simulink model "grid_forming_dqctrl"  (R2026b)
settings: Solver=VariableStepAuto
undefined symbols (not defined in the file or in its folder): param
libraries: nesl_utility x2, afe_ssc_lib x1
(part 1 of 2)
settings Model: Creator=d.bagnara  LastModifiedBy=dbagn

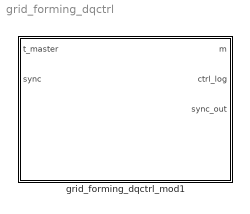
== system grid_forming_dqctrl ==
  grid_forming_dqctrl_mod1 : Subsystem  mask(Grid-forming AFE (two-level bridge, LCL filter)){p=param.afe_mod(1)}
      mask prompts: p "Parameter struct p (afe_module_param)"
      mask help: Grid-forming AFE in one block: ideal two-level bridge, DC-link capacitor and LCL filter as a Simscape language component (afe_ssc.afe_two_level_lcl), control and PWM as one MATLAB Function (afe_dq_ctrl_pwm, source private/afe_dq_ctrl_pwm.m of the library folder), measurements to the control through a Unit Delay of one tc (no algebraic loop). Interface of afe_dq_mod1 of grid_forming_dq.slx: ug_a/b/c left, Udc(+)/Udc(-) right, t_master in, M (17x1 pu) and ctrl_log (55x1) out. Master/slave: sync in and sync_out out, [theta; i_xi_ref; i_eta_ref; i_xi_n_ref; i_eta_n_ref]; with p.ctrl.slave = 1 the block runs its current loop with the angle and the current references of the master (sync_out of the master to sync of the slave), with p.ctrl.slave = 0 or absent it is a master and ignores sync. Negative-sequence compensator: p.ctrl.nsc_enable = 1 (same value in master and slaves) regulates the negative sequence of the terminal voltage to zero (PI in the negative frame, resonant term at 2*fgrid in the current loop); absent or 0, off. Open loop: p.ctrl.open_loop = 1 (same value in master and slaves) makes the block a V/f source without regulators, the voltage ug_ref at the angle of the phase generator as the EMF of the bridge (ol_udc_comp, ol_t_ramp); absent or 0, off. Droop: p.ctrl.droop = 1 makes the block a droop-controlled module for power sharing with other modules on the grid and in an island (P-f and Q-V droops, virtual impedance, voltage PI on the filter capacitor with feedforward, synchronization to the bus or black start; droop_* fields; sync then carries setpoint offsets [-; dP*; dQ*; dU*; dw*]); absent or 0, off. Parameter p: struct with the fields hw, pwm, ctrl, e.g. grid_forming_param_example.m of this folder (400 V, 250 kW, 50 Hz, 4 kHz) or param.afe_mod(1) of the study model. Description and user guide: the Help of this block (note library/documentation/grid_forming_following_afe).
      mask Help: eval('pwrdoc = which(''grid_forming_following_afe.pdf''); if isempty(pwrdoc), pwrdoc = ''https://github.com/pwr-control/library/blob/main/library/documentation/grid_forming_following_afe/grid_forming_following_afe.pdf''; end; web(pwrdoc, ''-browser''); clear pwrdoc')
      mask Display:
      | port_label('LConn', 1, 'ug_a');
      | port_label('LConn', 2, 'ug_b');
      | port_label('LConn', 3, 'ug_c');
      | port_label('RConn', 1, 'Udc(+)');
      | port_label('RConn', 2, 'Udc(-)');
      | port_label('input', 1, 't_master');
      | port_label('input', 2, 'sync');
      | port_label('output', 1, 'm');
      | port_label('output', 2, 'ctrl_log');
      | port_label('output', 3, 'sync_out');

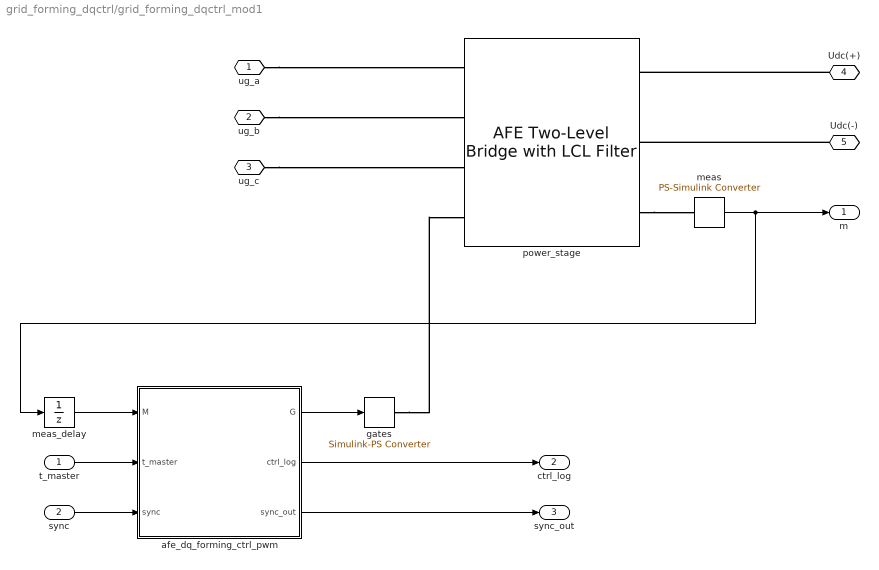
== system grid_forming_dqctrl/grid_forming_dqctrl_mod1 ==
  t_master : Inport
  sync : Inport  Port=2
  afe_dq_forming_ctrl_pwm : MATLAB Function  TreatAsAtomicUnit=on
  gates : nesl_utility/Simulink-PS Converter  PhysicalDomain=network_engine_domain  SubClassName=ps_input  LeftPortType=input  RightPortType=output  PseudoPeriodic=off  Frequencies=[]  NoiseDistribution=none  NoiseParameters=[]  Unit=V  AffineConversion=off  FilteringAndDerivatives=provide  SimscapeFilterOrder=1  InputFilterTimeConstant=0.001  UdotUserProvided=0
  meas : nesl_utility/PS-Simulink Converter  PhysicalDomain=network_engine_domain  SubClassName=ps_output  LeftPortType=input  RightPortType=output  PseudoPeriodic=off  Frequencies=[]  VectorFormat=inherit  Unit=1  AffineConversion=off
  meas_delay : UnitDelay  SampleTime=p.pwm.tc
  power_stage : afe_ssc_lib/AFE Two-Level Bridge with LCL Filter  Vth=p.hw.Vth V  Ron=p.hw.Ron Ohm  Goff=p.hw.Goff 1/Ohm  cap_dc=afe_ssc.onoff.on  Cdc=p.hw.Cdc F  Rdc=p.hw.Rdc Ohm  L1p=p.hw.L1p H  L10=p.hw.L10 H  R1=p.hw.R1 Ohm  Lls1=p.hw.Lls1 H  Cf=p.hw.Cf F  Rcf=p.hw.Rcf Ohm  L2p=p.hw.L2p H  L20=p.hw.L20 H  R2=p.hw.R2 Ohm  Lls2=p.hw.Lls2 H  ubez=p.hw.ubez V  ibez=p.hw.ibez A  udc_nom=p.hw.udc_nom V  vdc_specify=off  vdc_priority=None  vdc=0 V  vdc_nominal_specify=off  vdc_nominal_value=1  vdc_nominal_unit=V  vcap_specify=off  vcap_priority=None  vcap=0 V  vcap_nominal_specify=off  vcap_nominal_value=1  vcap_nominal_unit=V  ic_specify=off  ic_priority=None  ic=0 A  ic_nominal_specify=off  ic_nominal_value=1  ic_nominal_unit=A  vm_a_specify=off  vm_a_priority=None  vm_a=0 V  vm_a_nominal_specify=off  vm_a_nominal_value=1  vm_a_nominal_unit=V  vm_b_specify=off  vm_b_priority=None  vm_b=0 V  vm_b_nominal_specify=off  vm_b_nominal_value=1  vm_b_nominal_unit=V  vm_c_specify=off  vm_c_priority=None  vm_c=0 V  vm_c_nominal_specify=off  vm_c_nominal_value=1  vm_c_nominal_unit=V  i_ah_specify=off  i_ah_priority=None  i_ah=0 A  i_ah_nominal_specify=off  i_ah_nominal_value=1  i_ah_nominal_unit=A  i_al_specify=off  i_al_priority=None  i_al=0 A  i_al_nominal_specify=off  i_al_nominal_value=1  i_al_nominal_unit=A  i_bh_specify=off  i_bh_priority=None  i_bh=0 A  i_bh_nominal_specify=off  i_bh_nominal_value=1  i_bh_nominal_unit=A  i_bl_specify=off  i_bl_priority=None  i_bl=0 A  i_bl_nominal_specify=off  i_bl_nominal_value=1  i_bl_nominal_unit=A  i_ch_specify=off  i_ch_priority=None  i_ch=0 A  i_ch_nominal_specify=off  i_ch_nominal_value=1  i_ch_nominal_unit=A  i_cl_specify=off  i_cl_priority=None  i_cl=0 A  i_cl_nominal_specify=off  i_cl_nominal_value=1  i_cl_nominal_unit=A  i1_a_specify=off  i1_a_priority=None  i1_a=0 A  i1_a_nominal_specify=off  i1_a_nominal_value=1  i1_a_nominal_unit=A  i1_b_specify=off  i1_b_priority=None  i1_b=0 A  i1_b_nominal_specify=off  i1_b_nominal_value=1  i1_b_nominal_unit=A  i1_c_specify=off  i1_c_priority=None  i1_c=0 A  i1_c_nominal_specify=off  i1_c_nominal_value=1  i1_c_nominal_unit=A  vk_a_specify=off  vk_a_priority=None  vk_a=0 V  vk_a_nominal_specify=off  vk_a_nominal_value=1  vk_a_nominal_unit=V  vk_b_specify=off  vk_b_priority=None  vk_b=0 V  vk_b_nominal_specify=off  vk_b_nominal_value=1  vk_b_nominal_unit=V  vk_c_specify=off  vk_c_priority=None  vk_c=0 V  vk_c_nominal_specify=off  vk_c_nominal_value=1  vk_c_nominal_unit=V  vn_specify=off  vn_priority=None  vn=0 V  vn_nominal_specify=off  vn_nominal_value=1  vn_nominal_unit=V  vc_a_specify=off  vc_a_priority=None  vc_a=0 V  vc_a_nominal_specify=off  vc_a_nominal_value=1  vc_a_nominal_unit=V  vc_b_specify=off  vc_b_priority=None  vc_b=0 V  vc_b_nominal_specify=off  vc_b_nominal_value=1  vc_b_nominal_unit=V  vc_c_specify=off  vc_c_priority=None  vc_c=0 V  vc_c_nominal_specify=off  vc_c_nominal_value=1  vc_c_nominal_unit=V  i2_a_specify=off  i2_a_priority=None  i2_a=0 A  i2_a_nominal_specify=off  i2_a_nominal_value=1  i2_a_nominal_unit=A  i2_b_specify=off  i2_b_priority=None  i2_b=0 A  i2_b_nominal_specify=off  i2_b_nominal_value=1  i2_b_nominal_unit=A  i2_c_specify=off  i2_c_priority=None  i2_c=0 A  i2_c_nominal_specify=off  i2_c_nominal_value=1  i2_c_nominal_unit=A  j_ab_specify=off  j_ab_priority=None  j_ab=0 A  j_ab_nominal_specify=off  j_ab_nominal_value=1  j_ab_nominal_unit=A  j_bc_specify=off  j_bc_priority=None  j_bc=0 A  j_bc_nominal_specify=off  j_bc_nominal_value=1  j_bc_nominal_unit=A
  ug_a : PMIOPort  Side=Left
  ug_b : PMIOPort  Port=2  Side=Left
  ug_c : PMIOPort  Port=3  Side=Left
  Udc(+) : PMIOPort  Port=4  Side=Right
  Udc(-) : PMIOPort  Port=5  Side=Right
  m : Outport
  ctrl_log : Outport  Port=2
  sync_out : Outport  Port=3
  wires:
  t_master/1 -> afe_dq_forming_ctrl_pwm/2(t_master)
  meas/1 -> m/1, meas_delay/1
  meas_delay/1 -> afe_dq_forming_ctrl_pwm/1(M)
  afe_dq_forming_ctrl_pwm/1(G) -> gates/1
  afe_dq_forming_ctrl_pwm/2(ctrl_log) -> ctrl_log/1
  sync/1 -> afe_dq_forming_ctrl_pwm/3(sync)
  afe_dq_forming_ctrl_pwm/3(sync_out) -> sync_out/1
  connections:
  gates/RConn1 -- power_stage/LConn4
  power_stage/RConn3 -- meas/LConn1
  ug_a/RConn1 -- power_stage/LConn1
  ug_b/RConn1 -- power_stage/LConn2
  ug_c/RConn1 -- power_stage/LConn3
  Udc(+)/RConn1 -- power_stage/RConn1
  Udc(-)/RConn1 -- power_stage/RConn2
